simulink model "untitled_final_waveforms"  (R2023b)
settings: Solver=FixedStepDiscrete  StartTime=0.0  StopTime=0.3  FixedStep=1e-6  RelTol=1e-3
libraries: slpidlib x3, spsDCVoltageSourceLib x1, spsGroundLib x1, spsPermanentMagnetSynchronousMachineLib x1, spsThreePhaseVIMeasurementLib x1, spsUniversalBridgeLib x1, sps_lib x1
settings Model: Creator=zxw  LastModifiedBy=zxw

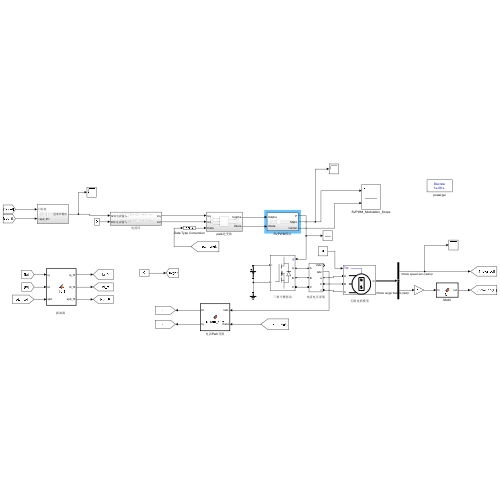
[thumbnail: Simulink's stored preview of the top-level diagram]
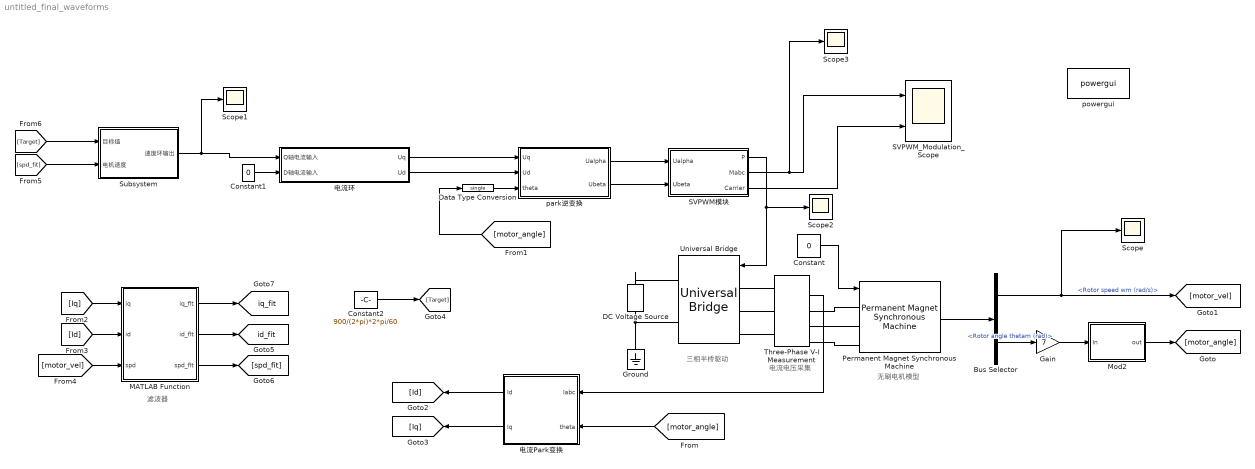
== system untitled_final_waveforms ==
  note: 滤波器
  note: 无刷电机模型
  note: 电流电压采集
  note: 三相半桥驱动
  Bus Selector : BusSelector  OutputSignals=Rotor speed wm (rad/s),Rotor angle thetam (rad)
  Constant : Constant  Value=0
  Constant1 : Constant  Value=0
  Constant2 : Constant  Value=900/(2*pi)*2*pi/60
  DC Voltage Source : spsDCVoltageSourceLib/DC Voltage Source  Amplitude=24  Measurements=None
  Data Type Conversion : DataTypeConversion  OutDataTypeStr=single  RndMeth=Nearest  SaturateOnIntegerOverflow=off
  Gain : Gain  Gain=7
  Ground : spsGroundLib/Ground  LConnTagsString=a
  MATLAB Function : MATLAB Function  TreatAsAtomicUnit=on
  Mod2 : MATLAB Function  TreatAsAtomicUnit=on
  Permanent Magnet Synchronous Machine : spsPermanentMagnetSynchronousMachineLib/Permanent Magnet Synchronous Machine  NbPhases=3  FluxDistribution=Sinusoidal  RotorType=Round  MechanicalLoad=Torque Tm  PresetModel=No  ShowDetailedParameters=on  MeasurementBus=off  Resistance=0.0485  Inductance=8.5e-3  dqInductances=[8.5e-3,8.5e-3]  La=0.000395  MachineConstant=Flux linkage established by magnets (V.s)  Flux=0.1194  VoltageCst=151.5974  TorqueCst=1.2537  Flat=120  Mechanical=[0.0027 0.0004924 7 0]  PolePairs=4  InitialConditions=[0,0, 0,0]  InitialConditions5ph=[0 0 0 0 0 0]  RefAngle=90 degrees behind phase A axis (modified Park)  IterativeDiscreteModel=Trapezoidal non iterative  TsBlock=-1  TsPowergui=0
  SVPWM_Modulation_Scope : Scope  NumInputPorts=2
  SVPWM模块 : Subsystem
  Scope{,1..3} (4 alike) : Scope
  Subsystem : Subsystem
  Three-Phase V-I Measurement : spsThreePhaseVIMeasurementLib/Three-Phase V-I Measurement  VoltageMeasurement=phase-to-ground  SetLabelV=off  LabelV=Vabc  Vpu=off  VpuLL=off  CurrentMeasurement=yes  SetLabelI=off  LabelI=Iabc  Ipu=off  Pbase=100e6  Vbase=500e3  OutputType=Complex  PhasorSimulation=off  PSBequivalent=0
  Universal Bridge : spsUniversalBridgeLib/Universal Bridge  Arms=3  SnubberResistance=1e5  SnubberCapacitance=inf  Device=MOSFET / Diodes  Ron=1e-3  Lon=0  ForwardVoltages="[  0  0  ]"  ForwardVoltage=0  GTOparameters=[ 10e-6 , 20e-6 ]  IGBTparameters=[ 1e-6 , 2e-6 ]  Measurements=None  Measurements_2=None  converterType=Rectifier
  park逆变换 : Subsystem
  powergui : sps_lib/powergui  Priority=1  SimulationMode=Discrete  SampleTime=1e-6  frequency=60  Iterations=50  frequencyindice=0  Pbase=100e6  ErrMax=1e-4  UnitsV=kV  UnitsW=MW  buscounter=0  FunctionMessages=off  echomessages=off  EnableUseOfTLC=off  CurrentSourceSwitches=off  DisableSnubberDevices=off  DisableRonSwitches=off  DisableVfSwitches=off  DisplayEquations=off  AutomaticDiscreteSolvers=off  SolverType=Tustin/Backward Euler (TBE)  Interpol=off  ExternalGateDelay=off  methode=off  Ts=100  x0status=blocks  SPID=on  SwTol=0  HookPort=off  NonlinearTolerance=1e-4  nMaxIteration=100  ContinueOnMaxIteration=off  RestoreLinks=warning  ResistiveCurrentMeasurement=off  Frange=[0:2:500]  Ylog=off  Xlog=on  ShowGrid=off  save=off  variable=ZData  structure=0  ZoomFFT=off  StartTime=0.0  cycles=1  DisplayStyle=1  fundamental=60  FreqAxis=off  MaxFrequency=1000  frequencyindicesteady=1  RmsSteady=1  display=off
  电流Park变换 : MATLAB Function  TreatAsAtomicUnit=on
  电流环 : Subsystem
  tag scope: id_fit=global, iq_fit=global
  wires:
  Permanent Magnet Synchronous Machine/1 -> Bus Selector/1
  Bus Selector/2 -> Gain/1  "<Rotor angle thetam (rad)>"
  Gain/1 -> Mod2/1(In)
  Mod2/1(out) -> [motor_angle]
  Bus Selector/1 -> Scope/1, [motor_vel]  "<Rotor speed wm (rad/s)>"
  Constant/1 -> Permanent Magnet Synchronous Machine/1
  park逆变换/2(Ubeta) -> SVPWM模块/2(Ubeta)
  park逆变换/1(Ualpha) -> SVPWM模块/1(Ualpha)
  Three-Phase V-I Measurement/2 -> 电流Park变换/1(Iabc)
  [motor_angle] -> 电流Park变换/2(theta)
  Data Type Conversion/1 -> park逆变换/3(theta)
  [motor_angle] -> Data Type Conversion/1
  电流Park变换/1(Id) -> [Id]
  电流Park变换/2(Iq) -> [Iq]
  [Iq] -> MATLAB Function/1(iq)
  [Id] -> MATLAB Function/2(id)
  [motor_vel] -> MATLAB Function/3(spd)
  MATLAB Function/1(iq_flt) -> [iq_fit]
  MATLAB Function/2(id_flt) -> [id_fit]
  MATLAB Function/3(spd_flt) -> [spd_fit]
  电流环/2(Ud) -> park逆变换/2(Ud)
  电流环/1(Uq) -> park逆变换/1(Uq)
  Constant1/1 -> 电流环/2(D轴电流输入)
  Constant2/1 -> [Target]
  [Target] -> Subsystem/1(目标值)
  [spd_fit] -> Subsystem/2(电机速度)
  Subsystem/1(速度环输出) -> Scope1/1, 电流环/1(Q轴电流输入)
  SVPWM模块/2(Mabc) -> Scope3/1, SVPWM_Modulation_Scope/1
  SVPWM模块/3(Carrier) -> SVPWM_Modulation_Scope/2
  SVPWM模块/1(P) -> Scope2/1, Universal Bridge/1
  connections:
  Three-Phase V-I Measurement/RConn1 -- Permanent Magnet Synchronous Machine/LConn1
  Three-Phase V-I Measurement/RConn2 -- Permanent Magnet Synchronous Machine/LConn2
  Three-Phase V-I Measurement/RConn3 -- Permanent Magnet Synchronous Machine/LConn3
  Universal Bridge/LConn1 -- Three-Phase V-I Measurement/LConn1
  Universal Bridge/LConn2 -- Three-Phase V-I Measurement/LConn2
  Universal Bridge/LConn3 -- Three-Phase V-I Measurement/LConn3
  DC Voltage Source/RConn1 -- Universal Bridge/RConn1
  DC Voltage Source/LConn1 -- Universal Bridge/RConn2 -- Ground/LConn1

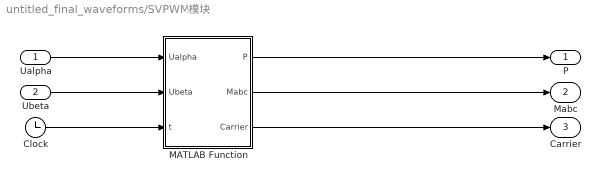
== system untitled_final_waveforms/SVPWM模块 ==
  Ualpha : Inport
  Ubeta : Inport  Port=2
  Clock : Clock
  MATLAB Function : MATLAB Function  TreatAsAtomicUnit=on
  P : Outport
  Mabc : Outport  Port=2
  Carrier : Outport  Port=3
  wires:
  Ualpha/1 -> MATLAB Function/1(Ualpha)
  MATLAB Function/1(P) -> P/1
  Ubeta/1 -> MATLAB Function/2(Ubeta)
  Clock/1 -> MATLAB Function/3(t)
  MATLAB Function/2(Mabc) -> Mabc/1
  MATLAB Function/3(Carrier) -> Carrier/1

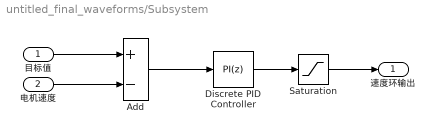
== system untitled_final_waveforms/Subsystem ==
  目标值 : Inport
  电机速度 : Inport  Port=2
  Add : Sum  Inputs=+-
  Discrete PID Controller : slpidlib/PID Controller  Controller=PI  Form=Parallel  TimeDomain=Discrete-time  UseExternalTs=off  SampleTime=1e-3  IntegratorMethod=Forward Euler  FilterMethod=Forward Euler  ControllerParametersSource=internal  P=0.334  I=14.88  UseKiTs=off  D=0  N=100  UseFilter=on  TunerSelectOption=Transfer Function Based (PID Tuner App)  InitialConditionSource=internal  InitialConditionForIntegrator=0  InitialConditionForFilter=0  DifferentiatorICPrevScaledInput=0  ExternalReset=none  TrackingMode=off  Kt=1  LimitOutput=on  SatLimitsSource=internal  UpperSaturationLimit=5  LowerSaturationLimit=-5  LinearizeAsGain=off  AntiWindupMode=back-calculation  Kb=50  LimitIntegrator=off  UpperIntegratorSaturationLimit=inf  LowerIntegratorSaturationLimit=-inf  POutMin=[]  POutMax=[]  IOutMin=[]  IOutMax=[]  DOutMin=[]  DOutMax=[]  NOutMin=[]  NOutMax=[]  SumOutMin=[]  SumOutMax=[]  SaturationOutMin=[]  SaturationOutMax=[]  PParamMin=[]  PParamMax=[]  IParamMin=[]  IParamMax=[]  DParamMin=[]  DParamMax=[]  NParamMin=[]  NParamMax=[]  KbParamMin=[]  KbParamMax=[]  KtParamMin=[]  KtParamMax=[]  KbOutMin=[]  KbOutMax=[]  KtOutMin=[]  KtOutMax=[]  IntegratorOutMin=[]  IntegratorOutMax=[]  FilterOutMin=[]  FilterOutMax=[]  SumI1OutMin=[]  SumI1OutMax=[]  SumI2OutMin=[]  SumI2OutMax=[]  SumI3OutMin=[]  SumI3OutMax=[]  SumI4OutMin=[]  SumI4OutMax=[]  SumDOutMin=[]  SumDOutMax=[]  DifferentiatorOutMin=[]  DifferentiatorOutMax=[]  FilterDiffOutCoefMin=[]  FilterDiffOutCoefMax=[]  ReciprocalOutMin=[]  ReciprocalOutMax=[]  SumDenOutMin=[]  SumDenOutMax=[]  SumNumOutMin=[]  SumNumOutMax=[]  DivideOutMin=[]  DivideOutMax=[]  UdiffTsProdOutMin=[]  UdiffTsProdOutMax=[]  NTsProdOutMin=[]  NTsProdOutMax=[]  UintegralTsProdOutMin=[]  UintegralTsProdOutMax=[]  UngainTsProdOutMin=[]  UngainTsProdOutMax=[]  ClampingZeroOutDataTypeStr=Inherit: Inherit via back propagation  ClampingZeroOutMin=[]  ClampingZeroOutMax=[]  FilterDenConstantOutDataTypeStr=Inherit: Inherit via back propagation  FilterDenConstantOutMin=[]  FilterDenConstantOutMax=[]  PCopyOutDataTypeStr=Inherit: Inherit via back propagation  PCopyOutMin=[]  PCopyOutMax=[]  NCopyOutDataTypeStr=Inherit: Inherit via back propagation  NCopyOutMin=[]  NCopyOutMax=[]  IntegratorContinuousStateAttributes=''  IntegratorStateMustResolveToSignalObject=off  IntegratorRTWStateStorageClass=Auto  FilterContinuousStateAttributes=''  FilterStateMustResolveToSignalObject=off  FilterRTWStateStorageClass=Auto  ParallelPVariant=InternalParameters  IdealPVariant=Disabled  IVariant=InternalParameters  DVariant=Disabled  IntegratorVariant=Discrete  SatVariant=Enabled  AWVariant=BackCalculation  PCopyVariant=Disabled  TRVariant=Disabled  FdbkBlocksVariant=Forward  IdealPFdbkVariant=Disabled  SatFdbkVariant=Disabled  DerivativeFilterVariant=Disabled  NVariant=Disabled  NCopyVariant=Disabled_SignalSpec  FilterICVariant=Disabled  IntegratorICVariant=InternalICs  ExternalResetVariant=Disabled  TRSumVariant=Passthrough  SumFdbkVariant=Disabled  SumVariant=Sum_PI  TsampFilterVariant=InternalTs  TsampNgainVariant=Passthrough  TsampIntegralVariant=Disabled_SignalSpec  ExternalSaturationOutDataTypeStr=Inherit: Same as second input
      settings: LibrarySourceBlock=simulink/Discrete/Discrete PID Controller
  Saturation : Saturate  UpperLimit=10  LowerLimit=-10
  速度环输出 : Outport
  wires:
  电机速度/1 -> Add/2
  目标值/1 -> Add/1
  Add/1 -> Discrete PID Controller/1
  Discrete PID Controller/1 -> Saturation/1
  Saturation/1 -> 速度环输出/1

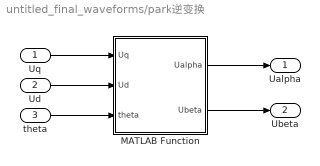
== system untitled_final_waveforms/park逆变换 ==
  Uq : Inport
  Ud : Inport  Port=2
  theta : Inport  Port=3
  MATLAB Function : MATLAB Function  TreatAsAtomicUnit=on
  Ualpha : Outport
  Ubeta : Outport  Port=2
  wires:
  MATLAB Function/1(Ualpha) -> Ualpha/1
  MATLAB Function/2(Ubeta) -> Ubeta/1
  Uq/1 -> MATLAB Function/1(Uq)
  Ud/1 -> MATLAB Function/2(Ud)
  theta/1 -> MATLAB Function/3(theta)

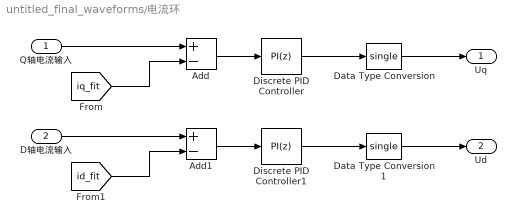
== system untitled_final_waveforms/电流环 ==
  Q轴电流输入 : Inport
  D轴电流输入 : Inport  Port=2
  Add : Sum  Inputs=+-
  Add1 : Sum  Inputs=+-
  Data Type Conversion : DataTypeConversion  OutDataTypeStr=single  RndMeth=Nearest  SaturateOnIntegerOverflow=off
  Data Type Conversion1 : DataTypeConversion  OutDataTypeStr=single  RndMeth=Nearest  SaturateOnIntegerOverflow=off
  Discrete PID Controller : slpidlib/PID Controller  Controller=PI  Form=Parallel  TimeDomain=Discrete-time  UseExternalTs=off  SampleTime=1e-4  IntegratorMethod=Forward Euler  FilterMethod=Forward Euler  ControllerParametersSource=internal  P=5.34  I=30.47  UseKiTs=off  D=0  N=100  UseFilter=on  TunerSelectOption=Transfer Function Based (PID Tuner App)  InitialConditionSource=internal  InitialConditionForIntegrator=0  InitialConditionForFilter=0  DifferentiatorICPrevScaledInput=0  ExternalReset=none  TrackingMode=off  Kt=1  LimitOutput=on  SatLimitsSource=internal  UpperSaturationLimit=24/sqrt(3)  LowerSaturationLimit=-24/sqrt(3)  LinearizeAsGain=off  AntiWindupMode=back-calculation  Kb=100  LimitIntegrator=off  UpperIntegratorSaturationLimit=inf  LowerIntegratorSaturationLimit=-inf  POutMin=[]  POutMax=[]  IOutMin=[]  IOutMax=[]  DOutMin=[]  DOutMax=[]  NOutMin=[]  NOutMax=[]  SumOutMin=[]  SumOutMax=[]  SaturationOutMin=[]  SaturationOutMax=[]  PParamMin=[]  PParamMax=[]  IParamMin=[]  IParamMax=[]  DParamMin=[]  DParamMax=[]  NParamMin=[]  NParamMax=[]  KbParamMin=[]  KbParamMax=[]  KtParamMin=[]  KtParamMax=[]  KbOutMin=[]  KbOutMax=[]  KtOutMin=[]  KtOutMax=[]  IntegratorOutMin=[]  IntegratorOutMax=[]  FilterOutMin=[]  FilterOutMax=[]  SumI1OutMin=[]  SumI1OutMax=[]  SumI2OutMin=[]  SumI2OutMax=[]  SumI3OutMin=[]  SumI3OutMax=[]  SumI4OutMin=[]  SumI4OutMax=[]  SumDOutMin=[]  SumDOutMax=[]  DifferentiatorOutMin=[]  DifferentiatorOutMax=[]  FilterDiffOutCoefMin=[]  FilterDiffOutCoefMax=[]  ReciprocalOutMin=[]  ReciprocalOutMax=[]  SumDenOutMin=[]  SumDenOutMax=[]  SumNumOutMin=[]  SumNumOutMax=[]  DivideOutMin=[]  DivideOutMax=[]  UdiffTsProdOutMin=[]  UdiffTsProdOutMax=[]  NTsProdOutMin=[]  NTsProdOutMax=[]  UintegralTsProdOutMin=[]  UintegralTsProdOutMax=[]  UngainTsProdOutMin=[]  UngainTsProdOutMax=[]  ClampingZeroOutDataTypeStr=Inherit: Inherit via back propagation  ClampingZeroOutMin=[]  ClampingZeroOutMax=[]  FilterDenConstantOutDataTypeStr=Inherit: Inherit via back propagation  FilterDenConstantOutMin=[]  FilterDenConstantOutMax=[]  PCopyOutDataTypeStr=Inherit: Inherit via back propagation  PCopyOutMin=[]  PCopyOutMax=[]  NCopyOutDataTypeStr=Inherit: Inherit via back propagation  NCopyOutMin=[]  NCopyOutMax=[]  IntegratorContinuousStateAttributes=''  IntegratorStateMustResolveToSignalObject=off  IntegratorRTWStateStorageClass=Auto  FilterContinuousStateAttributes=''  FilterStateMustResolveToSignalObject=off  FilterRTWStateStorageClass=Auto  ParallelPVariant=InternalParameters  IdealPVariant=Disabled  IVariant=InternalParameters  DVariant=Disabled  IntegratorVariant=Discrete  SatVariant=Enabled  AWVariant=BackCalculation  PCopyVariant=Disabled  TRVariant=Disabled  FdbkBlocksVariant=Forward  IdealPFdbkVariant=Disabled  SatFdbkVariant=Disabled  DerivativeFilterVariant=Disabled  NVariant=Disabled  NCopyVariant=Disabled_SignalSpec  FilterICVariant=Disabled  IntegratorICVariant=InternalICs  ExternalResetVariant=Disabled  TRSumVariant=Passthrough  SumFdbkVariant=Disabled  SumVariant=Sum_PI  TsampFilterVariant=InternalTs  TsampNgainVariant=Passthrough  TsampIntegralVariant=Disabled_SignalSpec  ExternalSaturationOutDataTypeStr=Inherit: Same as second input
      settings: LibrarySourceBlock=|
      | hdlsllib/HDL Floating Point
      | Operations/Discrete PID Controller
  Discrete PID Controller1 : slpidlib/PID Controller  Controller=PI  Form=Parallel  TimeDomain=Discrete-time  UseExternalTs=off  SampleTime=1e-4  IntegratorMethod=Forward Euler  FilterMethod=Forward Euler  ControllerParametersSource=internal  P=5.34  I=30.47  UseKiTs=off  D=0  N=100  UseFilter=on  TunerSelectOption=Transfer Function Based (PID Tuner App)  InitialConditionSource=internal  InitialConditionForIntegrator=0  InitialConditionForFilter=0  DifferentiatorICPrevScaledInput=0  ExternalReset=none  TrackingMode=off  Kt=1  LimitOutput=on  SatLimitsSource=internal  UpperSaturationLimit=24/sqrt(3)  LowerSaturationLimit=-24/sqrt(3)  LinearizeAsGain=off  AntiWindupMode=back-calculation  Kb=100  LimitIntegrator=off  UpperIntegratorSaturationLimit=inf  LowerIntegratorSaturationLimit=-inf  POutMin=[]  POutMax=[]  IOutMin=[]  IOutMax=[]  DOutMin=[]  DOutMax=[]  NOutMin=[]  NOutMax=[]  SumOutMin=[]  SumOutMax=[]  SaturationOutMin=[]  SaturationOutMax=[]  PParamMin=[]  PParamMax=[]  IParamMin=[]  IParamMax=[]  DParamMin=[]  DParamMax=[]  NParamMin=[]  NParamMax=[]  KbParamMin=[]  KbParamMax=[]  KtParamMin=[]  KtParamMax=[]  KbOutMin=[]  KbOutMax=[]  KtOutMin=[]  KtOutMax=[]  IntegratorOutMin=[]  IntegratorOutMax=[]  FilterOutMin=[]  FilterOutMax=[]  SumI1OutMin=[]  SumI1OutMax=[]  SumI2OutMin=[]  SumI2OutMax=[]  SumI3OutMin=[]  SumI3OutMax=[]  SumI4OutMin=[]  SumI4OutMax=[]  SumDOutMin=[]  SumDOutMax=[]  DifferentiatorOutMin=[]  DifferentiatorOutMax=[]  FilterDiffOutCoefMin=[]  FilterDiffOutCoefMax=[]  ReciprocalOutMin=[]  ReciprocalOutMax=[]  SumDenOutMin=[]  SumDenOutMax=[]  SumNumOutMin=[]  SumNumOutMax=[]  DivideOutMin=[]  DivideOutMax=[]  UdiffTsProdOutMin=[]  UdiffTsProdOutMax=[]  NTsProdOutMin=[]  NTsProdOutMax=[]  UintegralTsProdOutMin=[]  UintegralTsProdOutMax=[]  UngainTsProdOutMin=[]  UngainTsProdOutMax=[]  ClampingZeroOutDataTypeStr=Inherit: Inherit via back propagation  ClampingZeroOutMin=[]  ClampingZeroOutMax=[]  FilterDenConstantOutDataTypeStr=Inherit: Inherit via back propagation  FilterDenConstantOutMin=[]  FilterDenConstantOutMax=[]  PCopyOutDataTypeStr=Inherit: Inherit via back propagation  PCopyOutMin=[]  PCopyOutMax=[]  NCopyOutDataTypeStr=Inherit: Inherit via back propagation  NCopyOutMin=[]  NCopyOutMax=[]  IntegratorContinuousStateAttributes=''  IntegratorStateMustResolveToSignalObject=off  IntegratorRTWStateStorageClass=Auto  FilterContinuousStateAttributes=''  FilterStateMustResolveToSignalObject=off  FilterRTWStateStorageClass=Auto  ParallelPVariant=InternalParameters  IdealPVariant=Disabled  IVariant=InternalParameters  DVariant=Disabled  IntegratorVariant=Discrete  SatVariant=Enabled  AWVariant=BackCalculation  PCopyVariant=Disabled  TRVariant=Disabled  FdbkBlocksVariant=Forward  IdealPFdbkVariant=Disabled  SatFdbkVariant=Disabled  DerivativeFilterVariant=Disabled  NVariant=Disabled  NCopyVariant=Disabled_SignalSpec  FilterICVariant=Disabled  IntegratorICVariant=InternalICs  ExternalResetVariant=Disabled  TRSumVariant=Passthrough  SumFdbkVariant=Disabled  SumVariant=Sum_PI  TsampFilterVariant=InternalTs  TsampNgainVariant=Passthrough  TsampIntegralVariant=Disabled_SignalSpec  ExternalSaturationOutDataTypeStr=Inherit: Same as second input
      settings: LibrarySourceBlock=|
      | hdlsllib/HDL Floating Point
      | Operations/Discrete PID Controller
  Uq : Outport
  Ud : Outport  Port=2
  wires:
  Q轴电流输入/1 -> Add/1
  [iq_fit] -> Add/2
  D轴电流输入/1 -> Add1/1
  [id_fit] -> Add1/2
  Add/1 -> Discrete PID Controller/1
  Add1/1 -> Discrete PID Controller1/1
  Discrete PID Controller/1 -> Data Type Conversion/1
  Data Type Conversion/1 -> Uq/1
  Discrete PID Controller1/1 -> Data Type Conversion1/1
  Data Type Conversion1/1 -> Ud/1

== matlab function untitled_final_waveforms/SVPWM模块/MATLAB Function ==
  data: Ualpha input; P output; Ubeta input; t input; Mabc output; Carrier output
function [P, Mabc, Carrier] = spwm(Ualpha, Ubeta, t)
% SPWM三相桥驱动信号生成
%
% 输入：
%   Ualpha、Ubeta：alpha-beta坐标系参考电压，单位 V
%   t：仿真时间，单位 s
%
% 输出：
%   P：[A上 A下 B上 B下 C上 C下]'
%   Mabc：三相归一化调制波，范围 [-1, 1]
%   Carrier：双极性三角载波，范围 [-1, 1]

Vdc = 24;       % 直流母线电压
Fsw = 10000;    % 开关频率，10 kHz

%% SPWM线性范围限制
% SPWM最大参考电压矢量幅值为Vdc/2
Vlimit = 0.99*(Vdc/2);

% alpha-beta参考电压矢量幅值
Uref = sqrt(Ualpha*Ualpha + Ubeta*Ubeta);

% 对Ualpha和Ubeta等比例缩放
% 保持电压矢量方向不变，防止三相波形削顶
if Uref > Vlimit
    K = Vlimit/Uref;
    Ualpha = K*Ualpha;
    Ubeta  = K*Ubeta;
end

%% 逆Clarke变换：alpha-beta转三相参考电压
Va = Ualpha;
Vb = -0.5*Ualpha + sqrt(3)/2*Ubeta;
Vc = -0.5*Ualpha - sqrt(3)/2*Ubeta;

%% 三相归一化调制波
Mabc = zeros(3,1);

Mabc(1) = 2*Va/Vdc;
Mabc(2) = 2*Vb/Vdc;
Mabc(3) = 2*Vc/Vdc;

% 仅用于防止浮点数计算误差
Mabc(1) = min(max(Mabc(1), -1), 1);
Mabc(2) = min(max(Mabc(2), -1), 1);
Mabc(3) = min(max(Mabc(3), -1), 1);

%% 三相占空比
Da = 0.5*(Mabc(1) + 1);
Db = 0.5*(Mabc(2) + 1);
Dc = 0.5*(Mabc(3) + 1);

%% 生成中心对齐三角载波
% carrier范围为[0, 1]
carrierPhase = mod(t*Fsw, 1);
carrier = 1 - abs(2*carrierPhase - 1);

% 用于示波器显示的双极性载波
Carrier = 2*carrier - 1;

%% SPWM调制波与载波比较
Sa = double(Da >= carrier);
Sb = double(Db >= carrier);
Sc = double(Dc >= carrier);

%% 处理0%和100%占空比
if Da <= 0
    Sa = 0;
elseif Da >= 1
    Sa = 1;
end

if Db <= 0
    Sb = 0;
elseif Db >= 1
    Sb = 1;
end

if Dc <= 0
    Sc = 0;
elseif Dc >= 1
    Sc = 1;
end

%% 六路桥臂驱动信号
% 上下管互补，暂未加入死区时间
P = zeros(6,1);

P(1) = Sa;       % A相上管
P(2) = 1-Sa;     % A相下管

P(3) = Sb;       % B相上管
P(4) = 1-Sb;     % B相下管

P(5) = Sc;       % C相上管
P(6) = 1-Sc;     % C相下管
end

== matlab function untitled_final_waveforms/Mod2 ==
  data: In input; out output
function out = fcn(In)
out = mod(In, 2*pi);
end

== matlab function untitled_final_waveforms/park逆变换/MATLAB Function ==
  data: Uq input; Ualpha output; Ud input; theta input; Ubeta output
function [Ualpha, Ubeta] = inverse_park(Uq, Ud, theta)
% Inverse Park matching phase-a to q-axis convention
c = cos(theta);
s = sin(theta);
Ualpha = Uq*c + Ud*s;
Ubeta  = Uq*s - Ud*c;
end

== matlab function untitled_final_waveforms/电流Park变换 ==
  data: Iabc input; Id output; theta input; Iq output
function [Id, Iq] = current_park(Iabc, theta)
% Clarke + Park, phase-a aligned with q-axis
Ia = Iabc(1);
Ib = Iabc(2);
Ic = Iabc(3);
Ialpha = (2/3)*(Ia - 0.5*Ib - 0.5*Ic);
Ibeta  = (2/3)*(sqrt(3)/2)*(Ib - Ic);
c = cos(theta);
s = sin(theta);
Iq = Ialpha*c + Ibeta*s;
Id = Ialpha*s - Ibeta*c;
end

== matlab function untitled_final_waveforms/MATLAB Function ==
  settings: updateMethod=DISCRETE
  data: iq input; iq_flt output; id input; spd input; id_flt output; spd_flt output
function [iq_flt, id_flt, spd_flt] = filter3(iq, id, spd)
% iq、id和转速的一阶低通滤波器

% 实际执行周期
Ts = 1e-4;

% 截止频率
Fc_current = 2000;  % dq电流截止频率：2 kHz
Fc_speed   = 100;   % 转速截止频率：100 Hz

% 离散滤波系数
Alpha_current = 1 - exp(-2*pi*Fc_current*Ts);
Alpha_speed   = 1 - exp(-2*pi*Fc_speed*Ts);

% 滤波器内部状态
persistent iq_state id_state spd_state initialized

if isempty(initialized)
    % 使用第一次采样值初始化，避免启动跳变
    iq_state  = iq;
    id_state  = id;
    spd_state = spd;
    initialized = true;
end

% dq电流低通滤波
iq_state = iq_state + Alpha_current*(iq - iq_state);
id_state = id_state + Alpha_current*(id - id_state);

% 速度低通滤波
spd_state = spd_state + Alpha_speed*(spd - spd_state);

% 输出
iq_flt  = iq_state;
id_flt  = id_state;
spd_flt = spd_state;
end
